simulink model "Furuta_TorqueFuzzy_V2_Fix"  (R2025a)
settings: Solver=FixedStepDiscrete  StartTime=0  StopTime=30  FixedStep=0.001  RelTol=1e-3
model workspace (MAT data in the model file):
  Furuta_FuzzyPD25_Clean : mamfis (value not decoded)
libraries: fuzblock x1, mjLib x1
settings Model: Creator=vmano  LastModifiedBy=MINH TRÍ
settings OptimizationCC: ReuseModelBlockBuffer=off
settings ModelReferenceCC: EnableRefExpFcnMdlSchedulingChecks=on
settings SFSimCC: SimTargetLang=C++  SimDLTargetLibrary=mkl-dnn
settings RTWCC: GPUComputeCapability=3.5

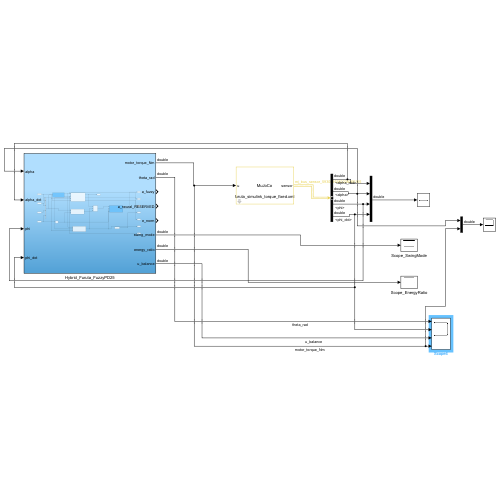
[thumbnail: Simulink's stored preview of the top-level diagram]
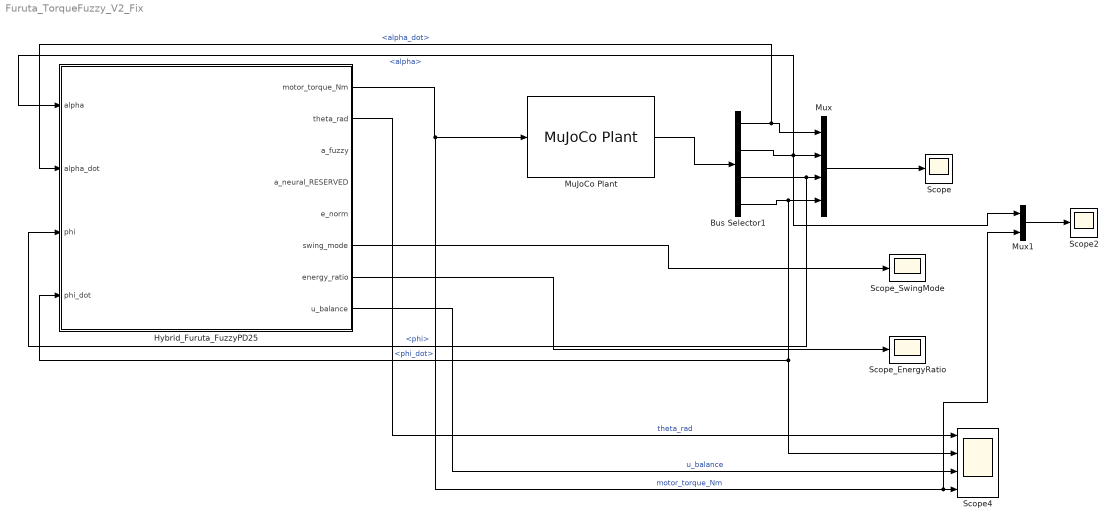
== system Furuta_TorqueFuzzy_V2_Fix ==
  Bus Selector1 : BusSelector  OutputSignals=alpha_dot,alpha,phi,phi_dot
  Hybrid_Furuta_FuzzyPD25 : Subsystem
  MuJoCo Plant : mjLib/MuJoCo Plant  controlBus=[]  sensorBus=mj_bus_sensor_7979902499018342666  controlLength=[]  sensorLength=[]  rgbLength=[]  depthLength=[]  sampleTime=0.001  xmlFileRel=C:\Furuta_MuJoCo\Furuta_SwingUpFix\furuta_simulink_torque_fixed.xml  xmlFile=C:\Furuta_MuJoCo\Furuta_SwingUpFix\furuta_simulink_torque_fixed.xml  renderingType=Global  vsync=off  visualFPS=60  zoomLevel=1  znear=0.001445  zfar=7.225  cameraSampleTime=0.020  rgbOutOption=on  depthOutOption=on  controlInterfaceType=Vector
      settings: SourceProductName=MuJoCo Simulator
  Mux : Mux
  Mux1 : Mux  Inputs=2
  Scope : Scope
      settings: ActiveDisplayYMinimum=-32.413204511153126  ActiveDisplayYMaximum=35.122833280536248
  Scope2 : Scope
      settings: ActiveDisplayYMinimum=-0.45385512110540166  ActiveDisplayYMaximum=1.987448633678623  DataLoggingVariableName=ScopeData2
  Scope4 : Scope  NumInputPorts=4
      settings: ActiveDisplayYMinimum=0.071974030763982511  ActiveDisplayYMaximum=0.79584061602317413  DataLoggingVariableName=ScopeData4
  Scope_EnergyRatio : Scope
      settings: ActiveDisplayYMinimum=-0.16035738231442129  ActiveDisplayYMaximum=1.4432164408297918
  Scope_SwingMode : Scope
      settings: ActiveDisplayYMinimum=-0.12499999999999997  ActiveDisplayYMaximum=1.125
  wires:
  MuJoCo Plant/1 -> Bus Selector1/1
  Bus Selector1/1 -> Hybrid_Furuta_FuzzyPD25/2(alpha_dot), Mux/1  "<alpha_dot>"
  Bus Selector1/2 -> Hybrid_Furuta_FuzzyPD25/1(alpha), Mux/2, Mux1/1  "<alpha>"
  Bus Selector1/3 -> Hybrid_Furuta_FuzzyPD25/3(phi), Mux/3  "<phi>"
  Bus Selector1/4 -> Scope4/2, Hybrid_Furuta_FuzzyPD25/4(phi_dot), Mux/4  "<phi_dot>"
  Mux/1 -> Scope/1
  Hybrid_Furuta_FuzzyPD25/1(motor_torque_Nm) -> Scope4/4, Mux1/2, MuJoCo Plant/1  "motor_torque_Nm"
  Hybrid_Furuta_FuzzyPD25/6(swing_mode) -> Scope_SwingMode/1
  Hybrid_Furuta_FuzzyPD25/7(energy_ratio) -> Scope_EnergyRatio/1
  Hybrid_Furuta_FuzzyPD25/8(u_balance) -> Scope4/3  "u_balance"
  Hybrid_Furuta_FuzzyPD25/2(theta_rad) -> Scope4/1  "theta_rad"
  Mux1/1 -> Scope2/1

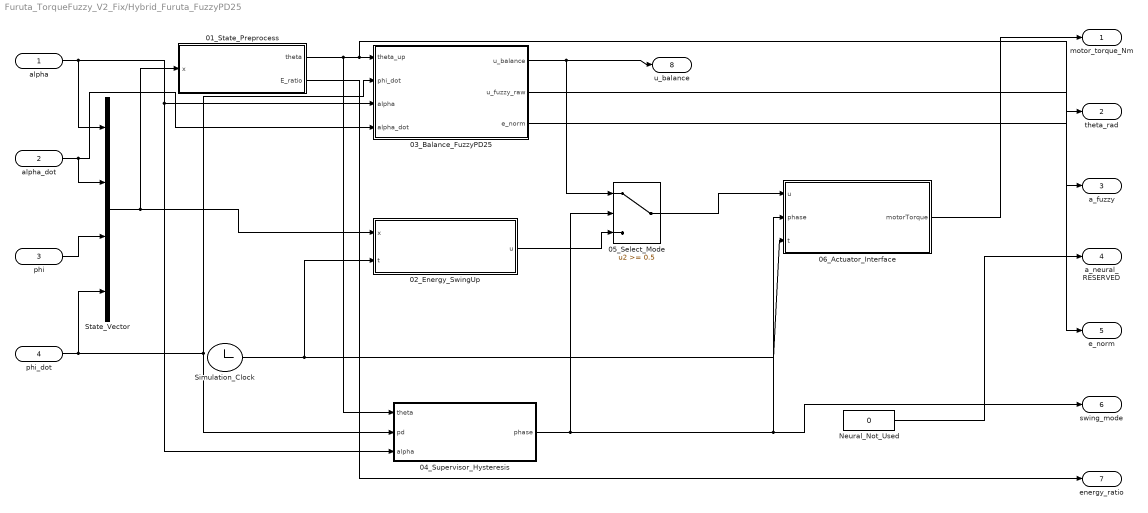
== system Furuta_TorqueFuzzy_V2_Fix/Hybrid_Furuta_FuzzyPD25 ==
  alpha : Inport
  alpha_dot : Inport  Port=2
  phi : Inport  Port=3
  phi_dot : Inport  Port=4
  01_State_Preprocess : MATLAB Function  TreatAsAtomicUnit=on
  02_Energy_SwingUp : MATLAB Function  TreatAsAtomicUnit=on
  03_Balance_FuzzyPD25 : Subsystem
  04_Supervisor_Hysteresis : MATLAB Function  TreatAsAtomicUnit=on
  05_Select_Mode : Switch  Threshold=0.5  SaturateOnIntegerOverflow=off  InputSameDT=off
  06_Actuator_Interface : MATLAB Function  TreatAsAtomicUnit=on
  Neural_Not_Used : Constant  Value=0
  Simulation_Clock : Clock
  State_Vector : Mux
  motor_torque_Nm : Outport
  theta_rad : Outport  Port=2
  a_fuzzy : Outport  Port=3
  a_neural_RESERVED : Outport  Port=4
  e_norm : Outport  Port=5
  swing_mode : Outport  Port=6
  energy_ratio : Outport  Port=7
  u_balance : Outport  Port=8
  wires:
  alpha/1 -> 03_Balance_FuzzyPD25/3(alpha), 04_Supervisor_Hysteresis/3(alpha), State_Vector/1
  alpha_dot/1 -> State_Vector/2, 03_Balance_FuzzyPD25/4(alpha_dot)
  phi/1 -> State_Vector/3
  phi_dot/1 -> 03_Balance_FuzzyPD25/2(phi_dot), 04_Supervisor_Hysteresis/2(pd), State_Vector/4
  State_Vector/1 -> 01_State_Preprocess/1(x), 02_Energy_SwingUp/1(x)
  Simulation_Clock/1 -> 02_Energy_SwingUp/2(t), 06_Actuator_Interface/3(t)
  01_State_Preprocess/1(theta) -> 03_Balance_FuzzyPD25/1(theta_up), theta_rad/1, 04_Supervisor_Hysteresis/1(theta)
  03_Balance_FuzzyPD25/1(u_balance) -> u_balance/1, 05_Select_Mode/1
  04_Supervisor_Hysteresis/1(phase) -> 06_Actuator_Interface/2(phase), swing_mode/1, 05_Select_Mode/2
  02_Energy_SwingUp/1(u) -> 05_Select_Mode/3
  05_Select_Mode/1 -> 06_Actuator_Interface/1(u)
  06_Actuator_Interface/1(motorTorque) -> motor_torque_Nm/1
  03_Balance_FuzzyPD25/2(u_fuzzy_raw) -> a_fuzzy/1
  Neural_Not_Used/1 -> a_neural_RESERVED/1
  03_Balance_FuzzyPD25/3(e_norm) -> e_norm/1
  01_State_Preprocess/2(E_ratio) -> energy_ratio/1

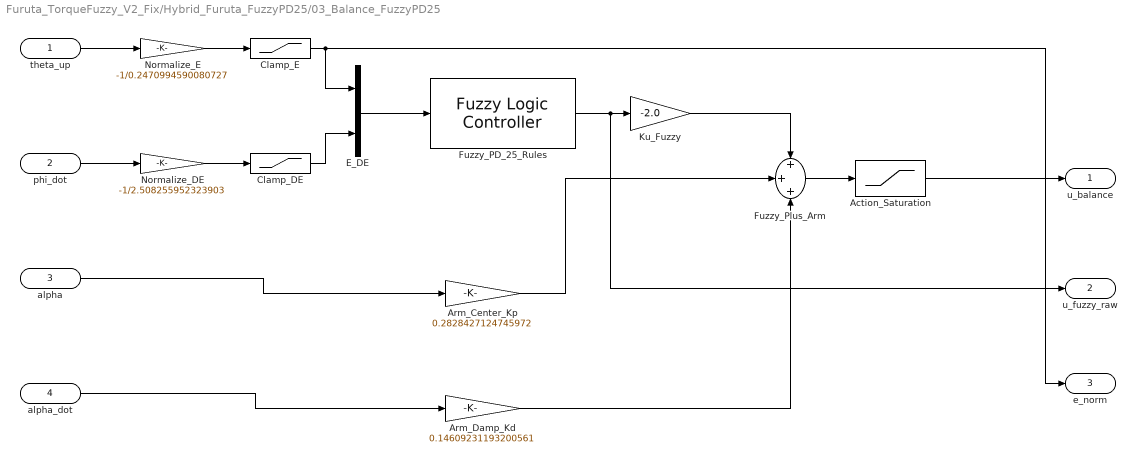
== system Furuta_TorqueFuzzy_V2_Fix/Hybrid_Furuta_FuzzyPD25/03_Balance_FuzzyPD25 ==
  theta_up : Inport
  phi_dot : Inport  Port=2
  alpha : Inport  Port=3
  alpha_dot : Inport  Port=4
  Action_Saturation : Saturate  UpperLimit=1  LowerLimit=-1
  Arm_Center_Kp : Gain  Gain=0.2828427124745972
  Arm_Damp_Kd : Gain  Gain=0.14609231193200561
  Clamp_DE : Saturate  UpperLimit=1  LowerLimit=-1
  Clamp_E : Saturate  UpperLimit=1  LowerLimit=-1
  E_DE : Mux  Inputs=2
  Fuzzy_PD_25_Rules : fuzblock/Fuzzy Logic  Controller  FIS=Furuta_FuzzyPD25_Clean  OutputSampleNumber=101  DataType=double  UseLookupTable=off  NumBreakpoints=10  FuzzifiedInputs=off  RuleFiringStrengths=off  RuleOutputs=off  AggregatedOutputs=off  SimulateUsing=Interpreted execution  OutOfRangeInputValueMessage=warning  NoRuleFiredMessage=warning  EmptyOutputFuzzySetMessage=warning
  Fuzzy_Plus_Arm : Sum  Inputs=+++
  Ku_Fuzzy : Gain  Gain=-2.0
  Normalize_DE : Gain  Gain=-1/2.508255952323903
  Normalize_E : Gain  Gain=-1/0.2470994590080727
  u_balance : Outport
  u_fuzzy_raw : Outport  Port=2
  e_norm : Outport  Port=3
  wires:
  theta_up/1 -> Normalize_E/1
  phi_dot/1 -> Normalize_DE/1
  Normalize_E/1 -> Clamp_E/1
  Normalize_DE/1 -> Clamp_DE/1
  Clamp_E/1 -> E_DE/1, e_norm/1
  Clamp_DE/1 -> E_DE/2
  E_DE/1 -> Fuzzy_PD_25_Rules/1
  Fuzzy_PD_25_Rules/1 -> Ku_Fuzzy/1, u_fuzzy_raw/1
  alpha/1 -> Arm_Center_Kp/1
  alpha_dot/1 -> Arm_Damp_Kd/1
  Ku_Fuzzy/1 -> Fuzzy_Plus_Arm/1
  Arm_Center_Kp/1 -> Fuzzy_Plus_Arm/2
  Arm_Damp_Kd/1 -> Fuzzy_Plus_Arm/3
  Fuzzy_Plus_Arm/1 -> Action_Saturation/1
  Action_Saturation/1 -> u_balance/1

== matlab function Furuta_TorqueFuzzy_V2_Fix/Hybrid_Furuta_FuzzyPD25/01_State_Preprocess ==
  data: x input; theta output; E_ratio output
function [theta, E_ratio] = fcn(x)
%#codegen
phi = x(3); pd = x(4);
theta = atan2(sin(phi-pi),cos(phi-pi));
m=0.014; l=0.051; Jp=8.06e-6+m*l*l; g=9.81;
E=0.5*Jp*pd*pd + m*g*l*(1-cos(phi));
E_ratio=E/(2*m*g*l);
end

== matlab function Furuta_TorqueFuzzy_V2_Fix/Hybrid_Furuta_FuzzyPD25/04_Supervisor_Hysteresis ==
  data: theta input; phase output; pd input; alpha input
function phase = fcn(theta,pd,alpha)
%#codegen
% 0=swing-up, 1=fuzzy balance. Separate capture/release thresholds.
persistent balanced
if isempty(balanced)
    balanced=false;
end
if balanced
    if abs(theta)>0.45 || abs(pd)>5.0 || abs(alpha)>2.1
        balanced=false;
    end
else
    if abs(theta)<0.25 && abs(pd)<2.5 && abs(alpha)<1.8
        balanced=true;
    end
end
phase=double(balanced);
end

== matlab function Furuta_TorqueFuzzy_V2_Fix/Hybrid_Furuta_FuzzyPD25/06_Actuator_Interface ==
  data: u input; motorTorque output; phase input; t input
function motorTorque = fcn(u,phase,t)
%#codegen
% Torque motor, gear=1, ctrlrange=[-0.010,0.010] N*m.
% phase and t remain as ports for compatibility with the supplied model.
% Both branches use the same torque scale; balance gains were tuned for it.
u=min(max(u,-1.0),1.0);
motorTorque=0.010*u;
end

== matlab function Furuta_TorqueFuzzy_V2_Fix/Hybrid_Furuta_FuzzyPD25/02_Energy_SwingUp ==
  data: x input; u output; t input
function u = fcn(x,t)
%#codegen
% Torque swing-up for the supplied MJCF, phi=0 DOWN, phi=pi UP.
% Output is normalized; the actuator interface multiplies by 0.010 N*m.
% State order: [alpha; alpha_dot; phi; phi_dot], all radians / rad/s.
alpha=x(1); ad=x(2); phi=x(3); pd=x(4);
m=0.014; l=0.051; R=0.065; g=9.81;
D=8.06e-6+m*l*l;
c=m*R*l;
b=8.06e-6+m*l*l-1e-7;
a0=1.05625e-5+0.03*0.035^2+m*R^2+1e-7;
mg=m*g*l;
sp=sin(phi); cp=cos(phi);

E=0.5*D*pd*pd+mg*(1-cp);
% An empirical swing-up energy margin for this model, not a new E_up.
energyError=1.5-E/(2*mg);
% Desired arm acceleration, with continuous centering and damping.
v=-30*energyError*pd*cp-40*alpha-12*ad;
if t<0.1
    v=v+20*sin(pi*t/0.1);
end
% Soft restoring action, without replacing the energy controller.
wall=max(abs(alpha)-1.5,0);
v=v-40*sign(alpha)*wall*wall;
v=min(max(v,-150),150);

% Partial feedback linearization: arm acceleration -> actual motor torque.
% M11=a0+b*sin(phi)^2, M12=c*cos(phi), M22=D.
M11=a0+b*sp*sp; M12=c*cp;
h1=2*b*sp*cp*ad*pd-c*sp*pd*pd;
h2=-b*sp*cp*ad*ad+mg*sp ...
   +9.899130726538984e-6*pd ...
   +1.846467096315846e-5*tanh(pd/0.01);
tau=(M11-M12*M12/D)*v+h1+0.0001*ad-M12*h2/D;
tau=min(max(tau,-0.010),0.010);
u=tau/0.010;
end
